simulink model "Quart_Car_Model_3"  (R2020b)
settings: Solver=VariableStepAuto  StartTime=0.0  StopTime=0.7  RelTol=1e-3
values from neighbouring files (symbols this model uses):
  Cs = 25    [Quart_Car_Script.m]
  Ct = 500    [Quart_Car_Script.m]
  Ks = 635    [Quart_Car_Script.m]
  Kt = 3000    [Quart_Car_Script.m]
  Ms = 0.435    [Quart_Car_Script.m]
  Mu = 0.119    [Quart_Car_Script.m]

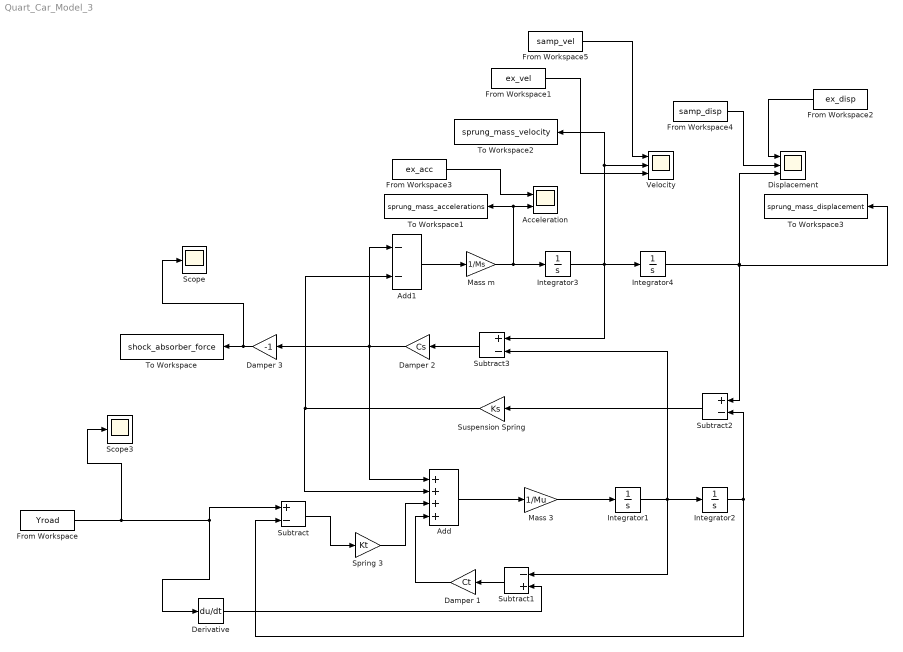
== system Quart_Car_Model_3 ==
  Acceleration : Scope  NumInputPorts=2
  Add : Sum  Inputs=++++
  Add1 : Sum  Inputs=--
  Damper 1 : Gain  Gain=Ct
  Damper 2 : Gain  Gain=Cs
  Damper 3 : Gain  Gain=-1
  Derivative : Derivative
  Displacement : Scope  NumInputPorts=3
  From Workspace : FromWorkspace  VariableName=Yroad  SampleTime=-1  OutputAfterFinalValue=Setting to zero
  From Workspace1 : FromWorkspace  VariableName=ex_vel  SampleTime=-1  OutputAfterFinalValue=Setting to zero
  From Workspace2 : FromWorkspace  VariableName=ex_disp  SampleTime=-1  OutputAfterFinalValue=Setting to zero
  From Workspace3 : FromWorkspace  VariableName=ex_acc  SampleTime=-1  OutputAfterFinalValue=Setting to zero
  From Workspace4 : FromWorkspace  VariableName=samp_disp  SampleTime=-1  OutputAfterFinalValue=Setting to zero
  From Workspace5 : FromWorkspace  VariableName=samp_vel  SampleTime=-1  OutputAfterFinalValue=Setting to zero
  Integrator{1..4} (4 alike) : Integrator
  Mass 3 : Gain  Gain=1/Mu
  Mass m : Gain  Gain=1/Ms
  Scope : Scope
  Scope3 : Scope
  Spring 3 : Gain  Gain=Kt
  Subtract : Sum  Inputs=+-
  Subtract1 : Sum  Inputs=-+
  Subtract2 : Sum  Inputs=+-
  Subtract3 : Sum  Inputs=+-
  Suspension Spring : Gain  Gain=Ks
  To Workspace : ToWorkspace  VariableName=shock_absorber_force  SaveFormat=Timeseries  SampleTime=-1
  To Workspace1 : ToWorkspace  VariableName=sprung_mass_accelerations  SaveFormat=Structure With Time  SampleTime=-1
  To Workspace2 : ToWorkspace  VariableName=sprung_mass_velocity  SaveFormat=Timeseries  SampleTime=-1
  To Workspace3 : ToWorkspace  VariableName=sprung_mass_displacement  SaveFormat=Timeseries  SampleTime=-1
  Velocity : Scope  NumInputPorts=3
  wires:
  Subtract/1 -> Spring 3/1
  Spring 3/1 -> Add/3
  Add/1 -> Mass 3/1
  Mass 3/1 -> Integrator1/1
  Integrator1/1 -> Subtract3/2, Subtract1/1, Integrator2/1
  Integrator2/1 -> Subtract/2, Subtract2/2
  Subtract1/1 -> Damper 1/1
  Damper 1/1 -> Add/4
  Subtract2/1 -> Suspension Spring/1
  Suspension Spring/1 -> Add1/2, Add/2
  Subtract3/1 -> Damper 2/1
  Damper 2/1 -> Damper 3/1, Add/1, Add1/1
  Add1/1 -> Mass m/1
  Mass m/1 -> To Workspace1/1, Acceleration/2, Integrator3/1
  Integrator3/1 -> Subtract3/1, To Workspace2/1, Velocity/2, Integrator4/1
  Integrator4/1 -> To Workspace3/1, Subtract2/1, Displacement/3
  Damper 3/1 -> Scope/1, To Workspace/1
  From Workspace/1 -> Scope3/1, Subtract/1, Derivative/1
  Derivative/1 -> Subtract1/2
  From Workspace1/1 -> Velocity/3
  From Workspace2/1 -> Displacement/1
  From Workspace3/1 -> Acceleration/1
  From Workspace4/1 -> Displacement/2
  From Workspace5/1 -> Velocity/1
